simulink model "ex_startup_load_step"  (R2026b)
settings: Solver=ode23t  StopTime=2  MaxStep=1e-4  RelTol=1e-5
undefined symbols (not defined in the file or in its folder): L1, L2, L3, Rechtsdrehfeld
libraries: asm_blocks_lib x17, nesl_utility x1
settings Model: Creator=fsbb  LastModifiedBy=fsbb
settings SimscapeCC: SimscapeLogType=all  SimscapeNominalValues="[{\"value\":\"1\",\"unit\":\"A\"},{\"value\":\"1\",\"unit\":\"bar\"},{\"value\":\"1\",\"unit\":\"cm^2\"},{\"value\":\"1\",\"unit\":\"cm^3/s\"},{\"value\":\"1\",\"unit\":\"kJ/kg\"},{\"value\":\"1\",\"unit\":\"kW\"},{\"value\":\"1\",\"unit\":\"l\"},{\"value\":\"1\",\"unit\":\"N\"},{\"value\":\"1\",\"unit\":\"N*m\"},{\"value\":\"1\",\"unit\":\"V\"},{\"value\":\"0.001\",\"unit\":\"Wb\"}]"  SimscapeUseEnergyAccounting=off

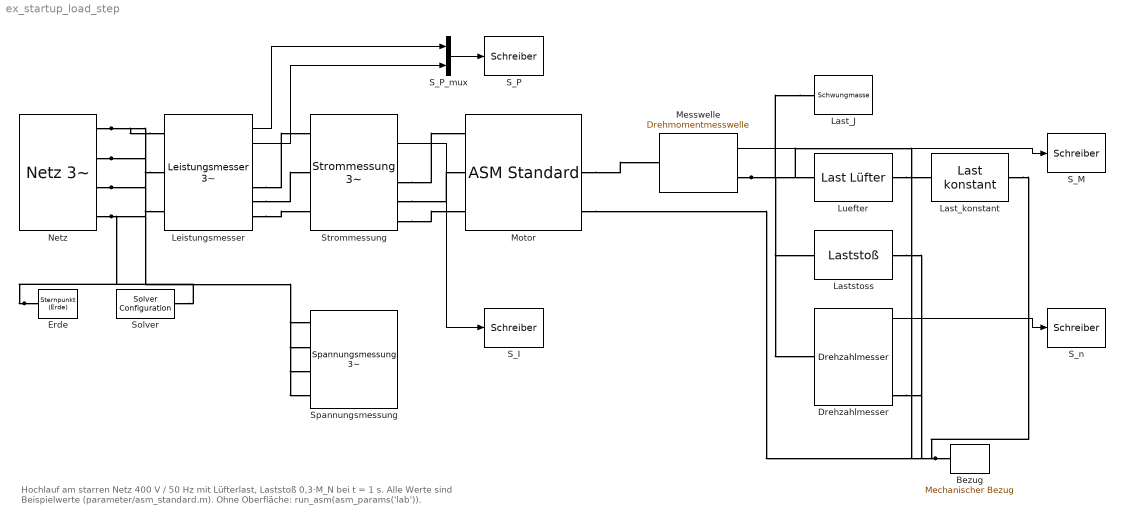
== system ex_startup_load_step ==
  note: Hochlauf am starren Netz 400 V / 50 Hz mit Lüfterlast, Laststoß 0,3·M_N bei t = 1 s. Alle Werte sind Beispielwerte (parameter/asm_standard.m). Ohne Oberfläche: run_asm(asm_params('lab')).
  Bezug : asm_blocks_lib/Mechanik/Mechanischer Bezug  Tag=asmlib:mech_reference
  Drehzahlmesser : asm_blocks_lib/Messgeräte/Drehzahlmesser  Tag=asmlib:speed_sensor  ns=1500
  Erde : asm_blocks_lib/Quellen/Sternpunkt (Erde)  Tag=asmlib:neutral_ground
  Last_J : asm_blocks_lib/Mechanik/Schwungmasse  Tag=asmlib:inertia  J=0.01  n0=0
  Last_konstant : asm_blocks_lib/Mechanik/Last konstant  Tag=asmlib:load_constant  M_L0=0
  Laststoss : asm_blocks_lib/Mechanik/Laststoß  Tag=asmlib:load_step  t_step=1  dM_L=7.95
  Leistungsmesser : asm_blocks_lib/Messgeräte/Leistungsmesser 3~  Tag=asmlib:power_meter3  f_meas=50
  Luefter : asm_blocks_lib/Mechanik/Last Lüfter  Tag=asmlib:load_fan  M_B=26.5  n_B=1440
  Messwelle : asm_blocks_lib/Messgeräte/Drehmomentmesswelle  Tag=asmlib:torque_sensor
  Motor : asm_blocks_lib/Maschine/ASM Standard  Tag=asmlib:asm_standard  param_set=Standard  connection=Stern  U_N=400  f_N=50  p=2  R1=0.5  L1s=0.009902  Lh=0.25  R2b=1.225  L2sb=0.009902  J_M=0.012  k_R=0  n0=0  l=0.15  r=0.06  N2=28  Bhat_N=0.8
  Netz : asm_blocks_lib/Quellen/Netz 3~  Tag=asmlib:grid3  U_L=400  f1=50  phase_seq=L1-L2-L3 (Rechtsdrehfeld)  phi0=0  t_on=0  R_N=0  L_N=0
  S_I : asm_blocks_lib/Messgeräte/Schreiber  Tag=asmlib:recorder  title_text=Strom (Effektivwert)
  S_M : asm_blocks_lib/Messgeräte/Schreiber  Tag=asmlib:recorder  title_text=Wellenmoment
  S_P : asm_blocks_lib/Messgeräte/Schreiber  Tag=asmlib:recorder  title_text=Wirk- und Blindleistung
  S_P_mux : Mux  Inputs=2
  S_n : asm_blocks_lib/Messgeräte/Schreiber  Tag=asmlib:recorder  title_text=Drehzahl
  Solver : nesl_utility/Solver Configuration  PhysicalDomain=network_engine_domain  SubClassName=solver  LeftPortType=input  RightPortType=generic  Tones=[]  Harmonics=[]  SimulateNoise=off  Profile=off  UseLocalSampling=off  EnableSwitchedLinearOptims=on  FrequencyDomain=off  UseCCode=off  RelTol=0.001  AbsTol=0.001  MinStep=1e-09  ToWorkspace=off  RevertToSquareIcSolve=off  NumHomotopyIterations=100  PhasorMode=off  PhasorModeNumHarmonics=1  ConsistencySolver=NEWTON_XTOL_AFTER_FTOL  CanonicalOrdering=CANONICAL  OptimizeIntermediates=OPTIMIZED  MulticoreSolverChoice=BACKWARD_EULER  IndexReductionMethod=DerivativeReplacement  DoDC=off  ResidualTolerance=1e-09  ConsistencyTolSource=GLOBAL  ConsistencyAbsTol=0.001  ConsistencyRelTol=0.001  ConsistencyTolFactor=0.001  UseLocalSolver=off  LocalSolverChoice=NE_BACKWARD_EULER_ADVANCER  ResolveIndetEquations=on  FunctionEvalNumThread=1  LocalSolverSampleTime=0.001  DoFixedCost=off  MaxNonlinIter=3  MaxModeIter=2  ComputeImpulses=off  ImpulseIterations=2  LinearAlgebra=auto  LinearAlgebraNumThread=0  EquationFormulation=NE_TIME_EF  DelaysMemoryBudget=1024  AutomaticFiltering=on  FilteringTimeConstant=0.001  PartitionStorageMethod=AS_NEEDED  PartitionMemoryBudget=1024  PartitionMethod=BALANCED  MultibodyUseLocalSolver=off  MultibodyLocalSolverChoice=ODE1  MultibodyLocalSolverSampleTime=0.001
  Spannungsmessung : asm_blocks_lib/Messgeräte/Spannungsmessung 3~  Tag=asmlib:voltage_sensor3  f_meas=50  reference=künstlicher Sternpunkt
  Strommessung : asm_blocks_lib/Messgeräte/Strommessung 3~  Tag=asmlib:current_sensor3  f_meas=50
  wires:
  Drehzahlmesser/1 -> S_n/1
  Messwelle/1 -> S_M/1
  Strommessung/2 -> S_I/1
  Leistungsmesser/1 -> S_P_mux/1
  Leistungsmesser/2 -> S_P_mux/2
  S_P_mux/1 -> S_P/1
  connections:
  Erde/LConn1 -- Netz/RConn4 -- Spannungsmessung/LConn4 -- Solver/RConn1
  Leistungsmesser/LConn1 -- Netz/RConn1 -- Spannungsmessung/LConn1
  Leistungsmesser/RConn1 -- Strommessung/LConn1
  Strommessung/RConn1 -- Motor/LConn1
  Leistungsmesser/LConn2 -- Netz/RConn2 -- Spannungsmessung/LConn2
  Leistungsmesser/RConn2 -- Strommessung/LConn2
  Strommessung/RConn2 -- Motor/LConn2
  Leistungsmesser/LConn3 -- Netz/RConn3 -- Spannungsmessung/LConn3
  Leistungsmesser/RConn3 -- Strommessung/LConn3
  Strommessung/RConn3 -- Motor/LConn3
  Motor/RConn1 -- Messwelle/LConn1
  Motor/RConn2 -- Luefter/RConn1 -- Laststoss/RConn1 -- Last_konstant/RConn1 -- Bezug/LConn1 -- Drehzahlmesser/RConn1
  Last_J/LConn1 -- Messwelle/RConn1 -- Luefter/LConn1 -- Laststoss/LConn1 -- Last_konstant/LConn1 -- Drehzahlmesser/LConn1
